simulink model "RLV4_elektromehanicki_OU"  (R2024b)
settings: Solver=VariableStepAuto  StartTime=0.0  StopTime=10.0  RelTol=1e-3
values from neighbouring files (symbols this model uses):
  b1 = 100    [skripta_zad1.m]
  b12 = 200    [skripta_zad1.m]
  b2 = 150    [skripta_zad1.m]
  k = 1e7    (= 10000000)    [skripta_zad1.m]
  kem = 20.28    [skripta_zad1.m]
  kme = 20.28    [skripta_zad1.m]
  L = 3.15e-3    (= 0.00315)    [skripta_zad1.m]
  m1 = 2    [skripta_zad1.m]
  m2 = 3    [skripta_zad1.m]
  R = 2.4    [skripta_zad1.m]
settings Model: Creator=stoja  LastModifiedBy=stoja

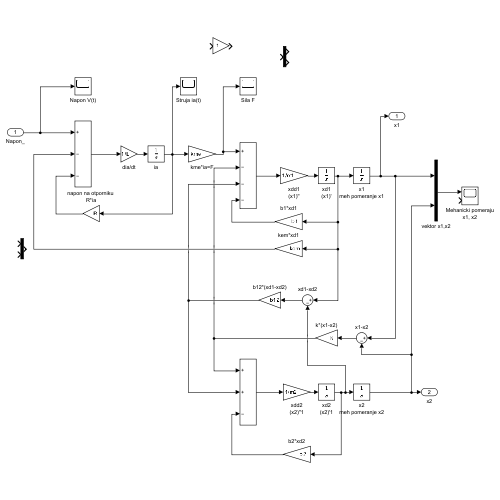
[thumbnail: Simulink's stored preview of the top-level diagram]
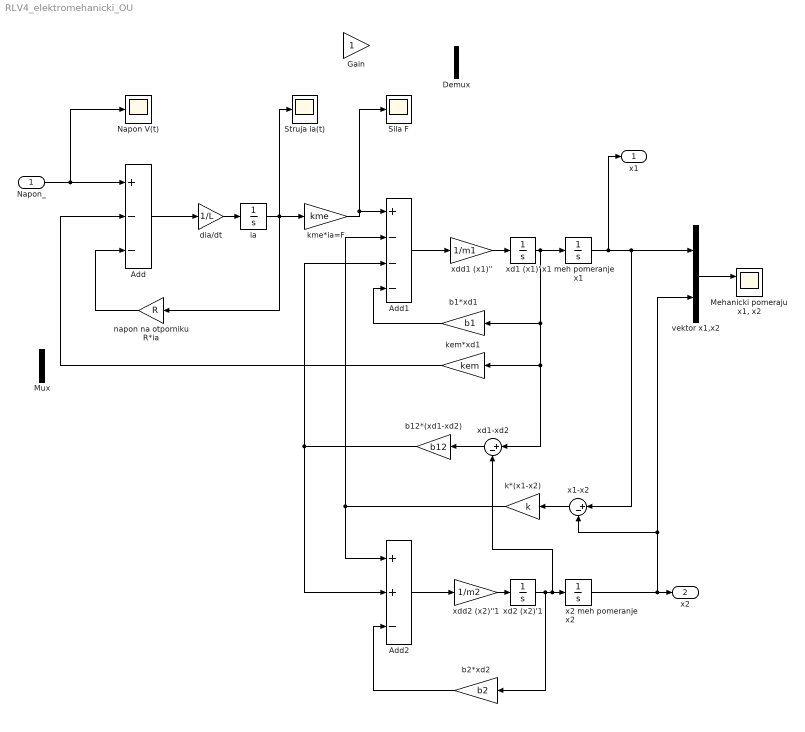
== system RLV4_elektromehanicki_OU ==
  Napon_ : Inport
  Add : Sum  Inputs=+--
  Add1 : Sum  Inputs=+---
  Add2 : Sum  Inputs=++-
  Demux : Demux  Outputs=2
  Gain : Gain
  "Mehanicki pomeraju x1, x2" : Scope  NumInputPorts=2
  Mux : Mux  Inputs=2
  Napon V(t) : Scope
  Sila F : Scope
  Struja ia(t) : Scope
  b1*xd1 : Gain  Gain=b1
  b12*(xd1-xd2) : Gain  Gain=b12
  b2*xd2 : Gain  Gain=b2
  dia/dt : Gain  Gain=1/L
  ia : Integrator
  k*(x1-x2) : Gain  Gain=k
  kem*xd1 : Gain  Gain=kem
  kme*ia=F : Gain  Gain=kme
  napon na otporniku R*ia : Gain  Gain=R
  vektor x1,x2 : Mux  Inputs=2
  x1 meh pomeranje x1 : Integrator
  x1-x2 : Sum  Inputs=|+-
  x2 meh pomeranje x2 : Integrator
  xd1 (x1)' : Integrator
  xd1-xd2 : Sum  Inputs=|+-
  xd2 (x2)'1 : Integrator
  xdd1 (x1)'' : Gain  Gain=1/m1
  xdd2 (x2)''1 : Gain  Gain=1/m2
  x1 : Outport
  x2 : Outport  Port=2
  wires:
  Napon_/1 -> Napon V(t)/1, Add/1
  Add/1 -> dia/dt/1
  dia/dt/1 -> ia/1
  ia/1 -> napon na otporniku R*ia/1, Struja ia(t)/1, kme*ia=F/1
  kme*ia=F/1 -> Sila F/1, Add1/1
  Add1/1 -> xdd1 (x1)''/1
  xdd1 (x1)''/1 -> xd1 (x1)'/1
  xd1 (x1)'/1 -> xd1-xd2/1, kem*xd1/1, b1*xd1/1, x1 meh pomeranje x1/1
  x1 meh pomeranje x1/1 -> vektor x1,x2/1, x1-x2/1, x1/1
  vektor x1,x2/1 -> "Mehanicki pomeraju x1, x2"/1
  napon na otporniku R*ia/1 -> Add/3
  kem*xd1/1 -> Add/2
  Add2/1 -> xdd2 (x2)''1/1
  xdd2 (x2)''1/1 -> xd2 (x2)'1/1
  xd2 (x2)'1/1 -> xd1-xd2/2, x2 meh pomeranje x2/1, b2*xd2/1
  b2*xd2/1 -> Add2/3
  x2 meh pomeranje x2/1 -> x1-x2/2, vektor x1,x2/2, x2/1
  x1-x2/1 -> k*(x1-x2)/1
  k*(x1-x2)/1 -> Add1/2, Add2/1
  xd1-xd2/1 -> b12*(xd1-xd2)/1
  b12*(xd1-xd2)/1 -> Add1/3, Add2/2
  b1*xd1/1 -> Add1/4
